simulink model "Ideal"  (R2022a)
settings: Solver=ode23tb  StartTime=0.0  StopTime=1  FixedStep=Ts  RelTol=1e-4
model workspace (MAT data in the model file):
  Ir1 = 900
  Ir2 = 300
  Ir3 = 250
  PMmpStc = 1005
  Pmmtstc = 1004.715
  T1 = 25
  T2 = 25
  T3 = 25
  initialDuty = 0.5
libraries: simulink x5, spsDiodeLib x4, spsSeriesRLCBranchLib x4, spsPVArrayLib x3, spsCurrentMeasurementLib x1, spsIGBTDiodeLib x1, spsPWMGeneratorDCDCLib x1, spsVoltageMeasurementLib x1, spspowerguiLib x1
settings Model: SimulationMode=accelerator  Creator=MathWorks  LastModifiedBy=archi
settings SolverCC: AlgebraicLoopSolver=LineSearch  SolverResetMethod=Robust
settings DataIOCC: LimitDataPoints=on  SaveFormat=Array  SignalLoggingSaveFormat=ModelDataLogs
settings OptimizationCC: ExpressionDepthLimit=2147483647  LifeSpan=inf
settings DebuggingCC: UnderspecifiedInitializationDetection=Classic  MergeDetectMultiDrivingBlocksExec=none  SolverPrmCheckMsg=warning  UnconnectedInputMsg=warning  UnconnectedOutputMsg=warning  UnconnectedLineMsg=warning  AllowSymbolicDim=off  StateNameClashWarn=warning  SFUnexpectedBacktrackingDiag=warning  SFNoUnconditionalDefaultTransitionDiag=warning  SFExecutionAtInitializationDiag=none  SFMachineParentedDataDiag=warning  ArithmeticOperatorsInVariantConditions=warning
settings HardwareCC: ProdBitPerPointer=32  ProdBitPerSizeT=32  ProdBitPerPtrDiffT=32  ProdLargestAtomicFloat=None  ProdIntDivRoundTo=Undefined  ProdEndianess=Unspecified  ProdWordSize=32  ProdHWDeviceType=32-bit Generic
settings ModelReferenceCC: PropagateSignalLabelsOutOfModel=off
settings SFSimCC: SimUseLocalCustomCode=off  CustomCodeUndefinedFunction=UseInterfaceOnly
settings RTWCC: RTWUseLocalCustomCode=off
settings CodeAppCC: StateflowObjectComments=on
settings GRTTargetCC: TargetLangStandard=C89/C90 (ANSI)  CombineOutputUpdateFcns=off  GRTInterface=on
settings ConfigComp: CovMetricSettings=dw  CovSaveCumulativeToWorkspaceVar=on  CovSaveSingleToWorkspaceVar=on  CovExternalEMLEnable=off  CovSFcnEnable=off
settings SimscapeCC: SimscapeNormalizeSystem=off

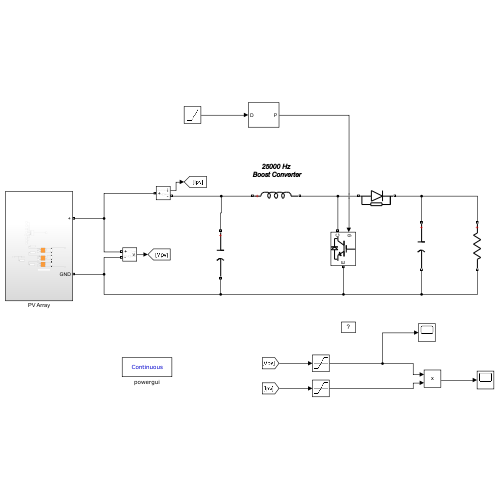
[thumbnail: Simulink's stored preview of the top-level diagram]
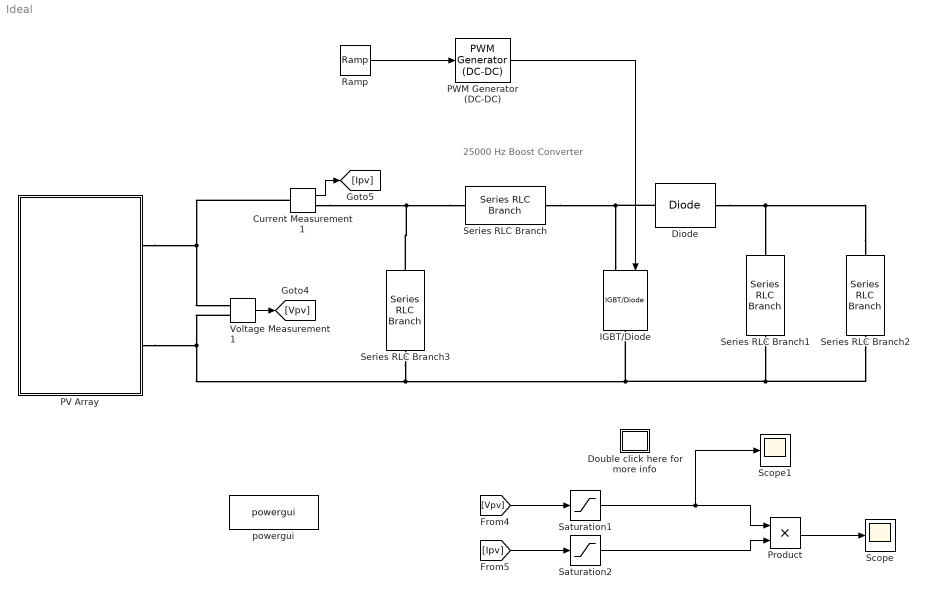
== system Ideal ==
  note: 25000 Hz
      | Boost Converter
  Current Measurement1 : spsCurrentMeasurementLib/Current Measurement  PhasorSimulation=off  OutputType=Complex  PSBequivalent=0
  Diode : spsDiodeLib/Diode  Ron=0.001  Lon=0  Vf=0.8  IC=0  UseSnubber=0  Rs=500  Cs=inf  Measurements=off
  Double click here for more info : Subsystem
      settings: OpenFcn=showdemo(bdroot(gcb))
      mask Display: disp('?')
  IGBT/Diode : spsIGBTDiodeLib/IGBT//Diode  Ron=1e-3  Rs=1e5  Cs=inf  Measurements=off
  PV Array : Subsystem
  PWM Generator (DC-DC) : spsPWMGeneratorDCDCLib/PWM Generator (DC-DC)  Fsw=25000  Ts=0
  Product : Product
  Ramp : simulink/Sources/Ramp  slope=1  start=0  InitialOutput=0
  Saturation1 : Saturate  UpperLimit=1000000000000000  LowerLimit=0
  Saturation2 : Saturate  UpperLimit=1000000000000000000  LowerLimit=0
  Scope : Scope
  Scope1 : Scope
  Series RLC Branch : spsSeriesRLCBranchLib/Series RLC Branch  LConnTagsString=__new0  RConnTagsString=__new0  BranchType=L  Resistance=1  Inductance=2.057e-3  SetiL0=off  InitialCurrent=0  Capacitance=1e-6  Setx0=off  InitialVoltage=0  Measurements=None
  Series RLC Branch1 : spsSeriesRLCBranchLib/Series RLC Branch  LConnTagsString=__new0  RConnTagsString=__new0  BranchType=C  Resistance=1  Inductance=1e-3  SetiL0=off  InitialCurrent=0  Capacitance=1.29e-05  Setx0=off  InitialVoltage=0  Measurements=None
  Series RLC Branch2 : spsSeriesRLCBranchLib/Series RLC Branch  LConnTagsString=__new0  RConnTagsString=__new0  BranchType=R  Resistance=61.71003717  Inductance=1e-3  SetiL0=off  InitialCurrent=0  Capacitance=1e-6  Setx0=off  InitialVoltage=0  Measurements=None
  Series RLC Branch3 : spsSeriesRLCBranchLib/Series RLC Branch  LConnTagsString=__new0  RConnTagsString=__new0  BranchType=C  Resistance=1e-4  Inductance=1.032e-3  SetiL0=off  InitialCurrent=0  Capacitance=3e-3  Setx0=off  InitialVoltage=0  Measurements=None
  Voltage Measurement1 : spsVoltageMeasurementLib/Voltage Measurement  PhasorSimulation=off  OutputType=Complex  PSBequivalent=0
  powergui : spspowerguiLib/powergui  Priority=1  SimulationMode=Continuous  SampleTime=0.00001  frequency=60  Iterations=50  frequencyindice=0  Pbase=100e6  ErrMax=1e-4  UnitsV=kV  UnitsW=MW  buscounter=0  FunctionMessages=off  echomessages=off  EnableUseOfTLC=off  CurrentSourceSwitches=on  DisableSnubberDevices=on  DisableRonSwitches=off  DisableVfSwitches=off  DisplayEquations=off  AutomaticDiscreteSolvers=off  SolverType=Tustin/Backward Euler (TBE)  Interpol=off  ExternalGateDelay=off  methode=off  Ts=0  x0status=blocks  SPID=off  SwTol=0  HookPort=off  NonlinearTolerance=1e-4  nMaxIteration=100  ContinueOnMaxIteration=off  RestoreLinks=warning  ResistiveCurrentMeasurement=off  Frange=[0:2:500]  Ylog=off  Xlog=on  ShowGrid=off  save=off  variable=ZData  structure=0  ZoomFFT=on  StartTime=0.0  cycles=1  DisplayStyle=1  fundamental=60  FreqAxis=off  MaxFrequency=1000  frequencyindicesteady=1  RmsSteady=1  display=off
  wires:
  Saturation1/1 -> Scope1/1, Product/1
  Current Measurement1/1 -> [Ipv]
  Voltage Measurement1/1 -> [Vpv]
  [Vpv] -> Saturation1/1
  [Ipv] -> Saturation2/1
  Saturation2/1 -> Product/2
  PWM Generator (DC-DC)/1 -> IGBT/Diode/1
  Product/1 -> Scope/1
  Ramp/1 -> PWM Generator (DC-DC)/1
  connections:
  Series RLC Branch2/LConn1 -- Diode/RConn1 -- Series RLC Branch1/LConn1
  Current Measurement1/LConn1 -- PV Array/RConn1 -- Voltage Measurement1/LConn1
  Series RLC Branch/LConn1 -- Series RLC Branch3/LConn1 -- Current Measurement1/RConn1
  PV Array/RConn2 -- Series RLC Branch2/RConn1 -- Series RLC Branch1/RConn1 -- IGBT/Diode/RConn1 -- Series RLC Branch3/RConn1 -- Voltage Measurement1/LConn2
  Series RLC Branch/RConn1 -- Diode/LConn1 -- IGBT/Diode/LConn1

== system Ideal/Double click here for more info ==

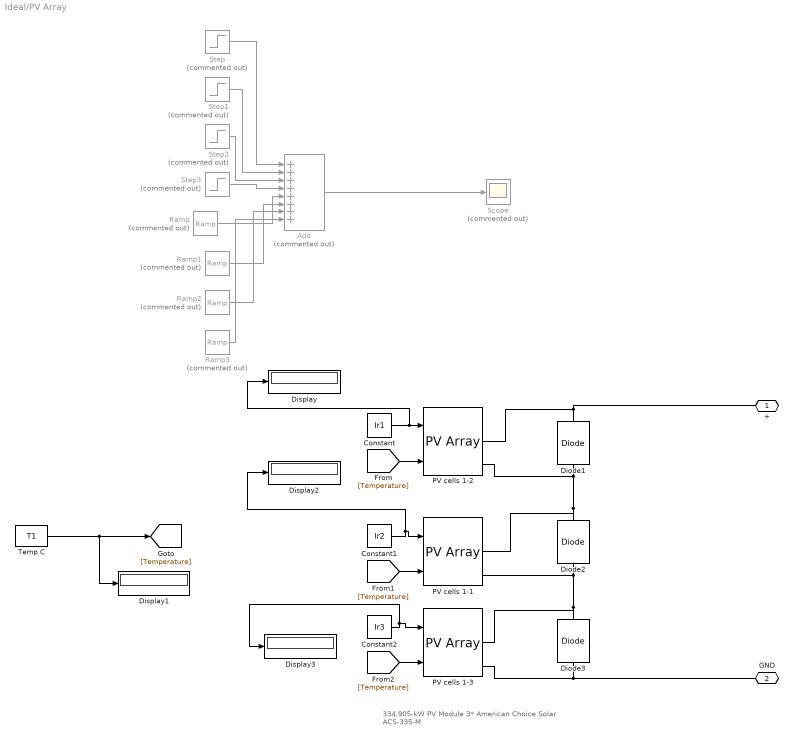
== system Ideal/PV Array ==
  note: 334.905-kW  PV Module
      | 3* American Choice Solar ACS-335-M
  Add : Sum  Commented=on  Inputs=++++++++
  Constant : Constant  Value=Ir1
  Constant1 : Constant  Value=Ir2
  Constant2 : Constant  Value=Ir3
  Diode1 : spsDiodeLib/Diode  Ron=0.001  Lon=0  Vf=0.7  IC=0  UseSnubber=off  Rs=1e5*inf  Cs=inf  Measurements=off
  Diode2 : spsDiodeLib/Diode  Ron=0.001  Lon=0  Vf=0.7  IC=0  UseSnubber=off  Rs=1e5*inf  Cs=inf  Measurements=off
  Diode3 : spsDiodeLib/Diode  Ron=0.001  Lon=0  Vf=0.7  IC=0  UseSnubber=off  Rs=1e5*inf  Cs=inf  Measurements=off
  Display{,1..3} (4 alike) : Display
  PV cells 1-1 : spsPVArrayLib/PV Array  Npar=1  Nser=1  PlotType=array @ 25 deg.C & specified irradiances  S_vec="[ 1000  500  100 ]"  Temp_C_vec="[ 45 25  ]"  ModuleName=User-defined  PlotWhenSelected=off  Pm=334.905  Ncell=80  Voc=49.9  Isc=9  Vm=41.5  Im=8.07  beta_Voc_pc=-0.36  alpha_Isc_pc=0.09  beta_Voc=-0.17964  alpha_Isc=0.0081  IL=9.0297  I0=3.1312e-10  nI=1.0111  Rsh=77.6407  Rs=0.25633  RobustModel=off  RobustCellTemperature=25  BAL=on  Tc=1e-5  Tfilter=5e-5
  PV cells 1-2 : spsPVArrayLib/PV Array  Npar=1  Nser=1  PlotType=array @ 1000 W/m2 & specified temperatures  S_vec="[ 1000  500  100 ]"  Temp_C_vec=[ 20 ]  ModuleName=User-defined  PlotWhenSelected=off  Pm=334.905  Ncell=80  Voc=49.9  Isc=9  Vm=41.5  Im=8.07  beta_Voc_pc=-0.36  alpha_Isc_pc=0.09  beta_Voc=-0.17964  alpha_Isc=0.0081  IL=9.0297  I0=3.1312e-10  nI=1.0111  Rsh=77.6407  Rs=0.25633  RobustModel=off  RobustCellTemperature=25  BAL=on  Tc=1e-5  Tfilter=5e-5
  PV cells 1-3 : spsPVArrayLib/PV Array  Npar=1  Nser=1  PlotType=array @ 25 deg.C & specified irradiances  S_vec="[ 1000  500  100 ]"  Temp_C_vec="[ 45 25  ]"  ModuleName=User-defined  PlotWhenSelected=off  Pm=334.905  Ncell=80  Voc=49.9  Isc=9  Vm=41.5  Im=8.07  beta_Voc_pc=-0.36  alpha_Isc_pc=0.09  beta_Voc=-0.17964  alpha_Isc=0.0081  IL=9.0297  I0=3.1312e-10  nI=1.0111  Rsh=77.6407  Rs=0.25633  RobustModel=off  RobustCellTemperature=25  BAL=on  Tc=1e-5  Tfilter=5e-5
  Ramp : simulink/Sources/Ramp  Commented=on  slope=100  start=2.3  InitialOutput=0
  Ramp1 : simulink/Sources/Ramp  Commented=on  slope=-100  start=4  InitialOutput=0
  Ramp2 : simulink/Sources/Ramp  Commented=on  slope=-100  start=5  InitialOutput=0
  Ramp3 : simulink/Sources/Ramp  Commented=on  slope=100  start=7  InitialOutput=0
  Scope : Scope  Commented=on
  Step : Step  Commented=on  Time=0  After=1000  SampleTime=0
  Step1 : Step  Commented=on  Time=0.6  After=-230  SampleTime=0
  Step2 : Step  Commented=on  After=-200  SampleTime=0
  Step3 : Step  Commented=on  Time=1.5  After=-200  SampleTime=0
  Temp C : Constant  Value=T1
  + : PMIOPort  Side=Right
  GND : PMIOPort  Port=2  Side=Right
  wires:
  Temp C/1 -> [Temperature], Display1/1
  Step/1 -> Add/1
  Step1/1 -> Add/2
  Step2/1 -> Add/3
  Step3/1 -> Add/4
  Ramp/1 -> Add/5
  Ramp1/1 -> Add/6
  Ramp2/1 -> Add/7
  Ramp3/1 -> Add/8
  Add/1 -> Scope/1
  Constant1/1 -> PV cells 1-1/1, Display2/1
  Constant2/1 -> PV cells 1-3/1, Display3/1
  Constant/1 -> PV cells 1-2/1, Display/1
  [Temperature] -> PV cells 1-2/2
  [Temperature] -> PV cells 1-1/2
  [Temperature] -> PV cells 1-3/2
  connections:
  PV cells 1-1/RConn1 -- Diode2/RConn1 -- PV cells 1-2/RConn2 -- Diode1/LConn1
  PV cells 1-2/RConn1 -- +/RConn1 -- Diode1/RConn1
  Diode2/LConn1 -- PV cells 1-3/RConn1 -- Diode3/RConn1 -- PV cells 1-1/RConn2
  PV cells 1-3/RConn2 -- GND/RConn1 -- Diode3/LConn1
